simulink model "su35_rebuild"  (R2025b)
settings: Solver=ode4  StartTime=0.0  StopTime=su35_stop_time  FixedStep=dt_fcs  RelTol=1e-3
values from neighbouring files (symbols this model uses):
  P = plant_get_params()    [make_rebuild_model.m]
undefined symbols (not defined in the file or in its folder): dt_fcs, su35_init
libraries: aerolibatmos2 x1, aerolibprivatev1p5 x1
settings Model: Creator=schultz  LastModifiedBy=schultz
settings DataIOCC: SaveOutput=off  SaveTime=off

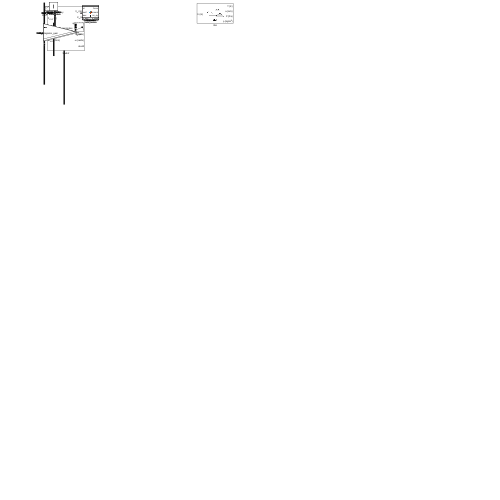
[thumbnail: Simulink's stored preview of the top-level diagram]
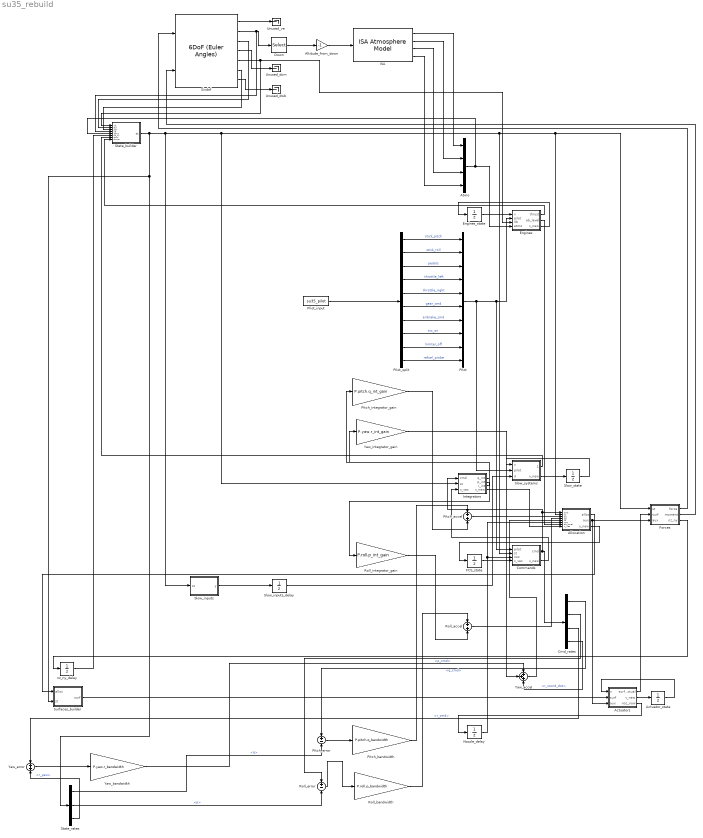
== system su35_rebuild ==
  Actuator_state : UnitDelay  InitialCondition=su35_init.actuators  SampleTime=dt_fcs  HasFrameUpgradeWarning=on
  Actuators : MATLAB Function  TreatAsAtomicUnit=on
  Allocation : MATLAB Function  TreatAsAtomicUnit=on
  Altitude_from_down : Gain  Gain=-1
  Atmo : Mux
  Cmd_rates : BusSelector  OutputSignals=q_cmd,p_cmd,r_cmd,r_coord_dot
  Commands : MATLAB Function  TreatAsAtomicUnit=on
  Down : Selector  InputPortWidth=3  IndexOptions=Index vector (dialog)  Indices=3  OutputSizes=1
  Engines : MATLAB Function  TreatAsAtomicUnit=on
  Engines_state : UnitDelay  InitialCondition=su35_init.engine  SampleTime=dt_fcs  HasFrameUpgradeWarning=on
  FCS_state : UnitDelay  InitialCondition=su35_init.fcs  SampleTime=dt_fcs  HasFrameUpgradeWarning=on
  Forces : MATLAB Function  TreatAsAtomicUnit=on
  ISA : aerolibatmos2/ISA Atmosphere Model  useExtended=off  action=None  custom=off  viscosityOut=off  g=9.80665  gamma=1.4  R=287.0531  L=0.0065  h_trop=11000  h_strat=20000  rho0=1.225  P0=101325  T0=288.15  h0=0  S=110.4  Tref=273.15  muref=1.716e-5
  Integrators : MATLAB Function  TreatAsAtomicUnit=on
  Nozzle_delay : UnitDelay  InitialCondition=su35_init.noz  SampleTime=dt_fcs  HasFrameUpgradeWarning=on
  Pilot : BusCreator  Inputs=10  OutDataTypeStr=Bus: Pilot
  Pilot_input : FromWorkspace  VariableName=su35_pilot  SampleTime=dt_fcs  Interpolate=off  OutputAfterFinalValue=Holding final value
  Pilot_split : Demux  Outputs=10
  Pitch_accel : Sum
  Pitch_bandwidth : Gain  Gain=P.pitch.q_bandwidth
  Pitch_error : Sum  Inputs=+-
  Pitch_integrator_gain : Gain  Gain=P.pitch.q_int_gain
  Roll_accel : Sum
  Roll_bandwidth : Gain  Gain=P.roll.p_bandwidth
  Roll_error : Sum  Inputs=+-
  Roll_integrator_gain : Gain  Gain=P.roll.p_int_gain
  Sixdof : aerolibprivatev1p5/6DoF (Euler Angles)  xme_0=su35_init.xme_0  Vm_0=su35_init.Vm_0  eul_0=su35_init.eul_0  pm_0=su35_init.pm_0  Mass=su35_init.mass  Inertia=su35_init.inertia
  Slow_inputs : MATLAB Function  TreatAsAtomicUnit=on
  Slow_inputs_delay : UnitDelay  InitialCondition=su35_init.slow_in  SampleTime=dt_fcs  HasFrameUpgradeWarning=on
  Slow_state : UnitDelay  InitialCondition=su35_init.slow  SampleTime=dt_fcs  HasFrameUpgradeWarning=on
  Slow_systems : MATLAB Function  TreatAsAtomicUnit=on
  State_builder : MATLAB Function  TreatAsAtomicUnit=on
  State_rates : BusSelector  OutputSignals=q,p,r_yaw
  Surfaces_builder : MATLAB Function  TreatAsAtomicUnit=on
  Unused_dcm : Terminator
  Unused_dwb : Terminator
  Unused_ve : Terminator
  Yaw_accel : Sum  Inputs=+++
  Yaw_bandwidth : Gain  Gain=P.yaw.r_bandwidth
  Yaw_error : Sum
  Yaw_integrator_gain : Gain  Gain=P.yaw.r_int_gain
  nz_ny_delay : UnitDelay  InitialCondition=su35_init.nz_ny  SampleTime=dt_fcs  HasFrameUpgradeWarning=on
  wires:
  Forces/3(nz_ny) -> nz_ny_delay/1
  Forces/2(moment) -> Sixdof/2
  Actuators/3(noz_now) -> Nozzle_delay/1
  Actuators/2(v_new) -> Actuator_state/1
  Actuators/1(surf_actual) -> Forces/2(surf)
  Cmd_rates/4 -> Yaw_accel/3  "<r_coord_dot>"
  Cmd_rates/3 -> Yaw_error/1  "<r_cmd>"
  Cmd_rates/1 -> Pitch_error/1  "<q_cmd>"
  Allocation/3(x_new) -> FCS_state/1
  Allocation/2(aux) -> Actuators/3(aux), Forces/3(aux)
  Allocation/1(alloc) -> Surfaces_builder/1(alloc)
  Slow_state/1 -> Slow_systems/1(v)
  Cmd_rates/2 -> Roll_error/1  "<p_cmd>"
  Yaw_accel/1 -> Allocation/5(rd)
  Actuator_state/1 -> Actuators/1(v)
  Pilot_split/2 -> Pilot/2  "stick_roll"
  Pilot_split/1 -> Pilot/1  "stick_pitch"
  Roll_integrator_gain/1 -> Roll_accel/2
  ISA/3 -> Atmo/3
  Pitch_bandwidth/1 -> Pitch_accel/1
  Pilot_split/5 -> Pilot/5  "throttle_right"
  Sixdof/2 -> Down/1, State_builder/4(xe)
  Roll_error/1 -> Roll_bandwidth/1
  Altitude_from_down/1 -> ISA/1
  Sixdof/6 -> State_builder/3(pqr)
  Pilot_split/8 -> Pilot/8  "tvc_on"
  Engines/1(thrust) -> State_builder/8(thrust)
  Integrators/4(x_new) -> Allocation/8(x_vec)
  Pilot_input/1 -> Pilot_split/1
  Down/1 -> Altitude_from_down/1
  Integrators/2(p_int) -> Roll_integrator_gain/1
  Slow_inputs_delay/1 -> Slow_systems/3(st_prev)
  Pilot_split/4 -> Pilot/4  "throttle_left"
  Surfaces_builder/1(surf) -> Actuators/2(surf)
  Engines/2(ab_level) -> Allocation/7(ab_level)
  Slow_systems/1(slow_now) -> State_builder/7(slow)
  Commands/2(x_new) -> Integrators/3(x_vec)
  Sixdof/7 -> Unused_dwb/1
  Yaw_bandwidth/1 -> Yaw_accel/1
  State_rates/1 -> Pitch_error/2  "<q>"
  Roll_accel/1 -> Allocation/4(pd)
  Pilot_split/6 -> Pilot/6  "gear_cmd"
  State_rates/3 -> Yaw_error/2  "<r_yaw>"
  Pilot_split/3 -> Pilot/3  "pedals"
  State_builder/1(st) -> Surfaces_builder/2(st), State_rates/1, Forces/1(st), Allocation/2(st), Commands/2(st), Integrators/2(st), Slow_inputs/1(st)
  Pitch_integrator_gain/1 -> Pitch_accel/2
  Slow_systems/2(v_new) -> Slow_state/1
  ISA/4 -> Atmo/4
  nz_ny_delay/1 -> State_builder/6(nz_ny)
  Sixdof/1 -> Unused_ve/1
  Sixdof/5 -> Engines/3(Vb), State_builder/1(Vb)
  Slow_inputs/1(y) -> Slow_inputs_delay/1
  FCS_state/1 -> Commands/4(x_vec)
  Yaw_error/1 -> Yaw_bandwidth/1
  Sixdof/4 -> Unused_dcm/1
  Roll_bandwidth/1 -> Roll_accel/1
  ISA/2 -> Atmo/2
  Pitch_error/1 -> Pitch_bandwidth/1
  Pilot_split/7 -> Pilot/7  "airbrake_cmd"
  Pilot_split/9 -> Pilot/9  "limiter_off"
  State_rates/2 -> Roll_error/2  "<p>"
  Sixdof/3 -> State_builder/2(eul)
  Pilot_split/10 -> Pilot/10  "refuel_probe"
  Commands/1(cmd) -> Allocation/1(cmd), Integrators/1(cmd), Cmd_rates/1
  Yaw_integrator_gain/1 -> Yaw_accel/2
  Engines_state/1 -> Engines/1(v)
  Atmo/1 -> Engines/4(atmo), State_builder/5(atmo)
  Integrators/3(r_int) -> Yaw_integrator_gain/1
  Pilot/1 -> Commands/1(pilot), Engines/2(pilot), Slow_systems/2(pilot)
  Integrators/1(q_int) -> Pitch_integrator_gain/1
  Forces/1(force) -> Sixdof/1
  Pitch_accel/1 -> Allocation/3(qd)
  Nozzle_delay/1 -> Commands/3(noz), Allocation/6(noz)
  ISA/1 -> Atmo/1
  Engines/3(v_new) -> Engines_state/1

== matlab function su35_rebuild/Actuators ==
  data: v input; surf_actual output Bus: Surfaces; surf input Bus: Surfaces; aux input Bus: Aux; v_new output; noz_now output
function [surf_actual, v_new, noz_now] = f(v, surf, aux)
P = coder.const(plant_get_params());
[surf_actual, v_new, noz_now] = plant_actuators_step(P, v, surf, aux, 0.006);
end

== matlab function su35_rebuild/Forces ==
  data: st input Bus: State; force output; surf input Bus: Surfaces; aux input Bus: Aux; moment output; nz_ny output
function [force, moment, nz_ny] = f(st, surf, aux)
P = coder.const(plant_get_params());
[force, moment, nz_ny] = plant_step_forces(P, st, surf, aux);
end

== matlab function su35_rebuild/Engines ==
  data: v input; thrust output; pilot input Bus: Pilot; Vb input; atmo input; ab_level output; v_new output
function [thrust, ab_level, v_new] = f(v, pilot, Vb, atmo)
P = coder.const(plant_get_params());
[thrust, ab_level, v_new] = plant_engines_step(P, v, pilot, Vb, atmo, 0.006);
end

== matlab function su35_rebuild/State_builder ==
  data: Vb input; st output Bus: State; eul input; pqr input; xe input; atmo input; nz_ny input; slow input; thrust input
function st = f(Vb, eul, pqr, xe, atmo, nz_ny, slow, thrust)
P = coder.const(plant_get_params());
st = plant_make_state(P, Vb, eul, pqr, xe, atmo, nz_ny, slow, thrust);
end

== matlab function su35_rebuild/Slow_systems ==
  data: v input; slow_now output; pilot input Bus: Pilot; st_prev input; v_new output
function [slow_now, v_new] = f(v, pilot, st_prev)
P = coder.const(plant_get_params());
[slow_now, v_new] = plant_slow_vec_step(P, v, pilot, st_prev, 0.006);
end

== matlab function su35_rebuild/Slow_inputs ==
  data: st input Bus: State; y output
function y = f(st)
y = [st.mach; st.alpha; st.nz; st.qbar];
end

== matlab function su35_rebuild/Commands ==
  data: pilot input Bus: Pilot; cmd output Bus: FcsCmd; st input Bus: State; noz input; x_vec input; x_new output
function [cmd, x_new] = f(pilot, st, noz, x_vec)
P = coder.const(plant_get_params());
x = fcs_state_unpack(x_vec);
[cmd, x] = fcs_commands(P, pilot, st, noz(1), x, 0.006);
x_new = fcs_state_pack(x);
end

== matlab function su35_rebuild/Integrators ==
  data: cmd input Bus: FcsCmd; q_int output; st input Bus: State; x_vec input; p_int output; r_int output; x_new output
function [q_int, p_int, r_int, x_new] = f(cmd, st, x_vec)
P = coder.const(plant_get_params());
x = fcs_state_unpack(x_vec);
[q_int, p_int, r_int, x] = fcs_integrators(P, cmd, st, x, 0.006);
x_new = fcs_state_pack(x);
end

== matlab function su35_rebuild/Allocation ==
  data: cmd input Bus: FcsCmd; alloc output Bus: AllocOut; st input Bus: State; qd input; pd input; rd input; noz input; ab_level input; x_vec input; aux output Bus: Aux; x_new output
function [alloc, aux, x_new] = f(cmd, st, qd, pd, rd, noz, ab_level, x_vec)
P = coder.const(plant_get_params());
x = fcs_state_unpack(x_vec);
act.noz_pitch = noz(1);
act.noz_yaw = noz(2);
[alloc, aux, x] = fcs_allocation(P, cmd, st, qd, pd, rd, act, ab_level, x, 0.006);
x_new = fcs_state_pack(x);
end

== matlab function su35_rebuild/Surfaces_builder ==
  data: alloc input Bus: AllocOut; surf output Bus: Surfaces; st input Bus: State
function surf = f(alloc, st)
P = coder.const(plant_get_params());
surf = fcs_surfaces(P, alloc, st);
end
